simulink model "TP6_Verifcation_intervalle_avec_variables_locales"  (R2022b)
settings: Solver=VariableStepAuto  StartTime=0.0  StopTime=inf  RelTol=1e-3
settings Model: Creator=LENOVO  LastModifiedBy=HP
settings OptimizationCC: ReuseModelBlockBuffer=on
settings RTWCC: GPUComputeCapability=5.0

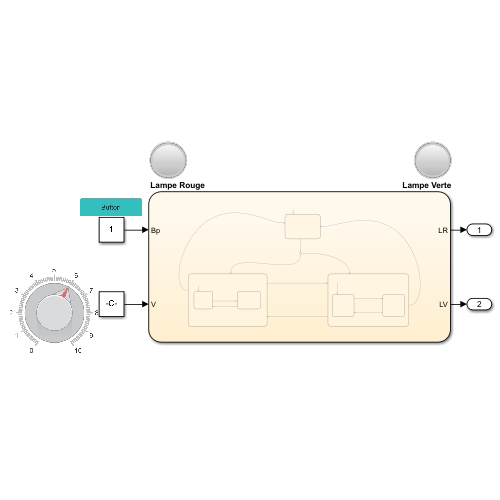
[thumbnail: Simulink's stored preview of the top-level diagram]
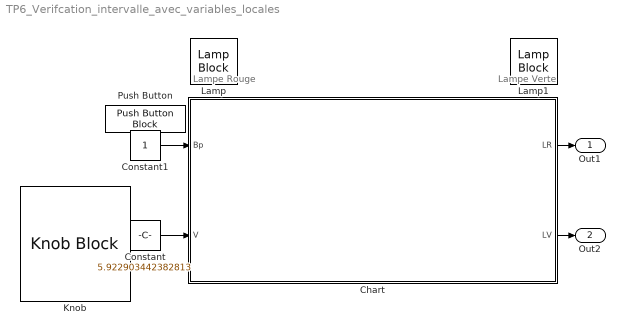
== system TP6_Verifcation_intervalle_avec_variables_locales ==
  note: Lampe Rouge
  note: Lampe Verte
  Chart : Stateflow chart  TreatAsAtomicUnit=on
  Constant : Constant  Value=5.922903442382813
  Constant1 : Constant
  Knob : KnobBlock  LabelPosition=Hide  ScaleMax=10
  Lamp : LampBlock  LabelPosition=Hide
  Lamp1 : LampBlock  LabelPosition=Hide
  Push Button : PushButtonBlock  ButtonType=Latch  OffValue=0.000000
  Out1 : Outport
  Out2 : Outport  Port=2
  wires:
  Constant1/1 -> Chart/1(Bp)
  Constant/1 -> Chart/2(V)
  Chart/1(LR) -> Out1/1
  Chart/2(LV) -> Out2/1

== stateflow chart TP6_Verifcation_intervalle_avec_variables_locales/Chart ==
  state initial
    entry:
    LV=0;
    LR=0;
  state plage_valide
    state on
      entry:
      LV=0;
      LR=1;
    state off
      entry:
      LV=0;
      LR=0;
    (default) -> plage_valide.on
    plage_valide.on -> plage_valide.off : [after (0.5, sec)]
    plage_valide.off -> plage_valide.on : [after (0.5, sec)]
  state plage_invalide
    state on
      entry:
      LV=1;
      LR=0;
    state off
      entry:
      LV=0;
      LR=0;
    (default) -> plage_invalide.on
    plage_invalide.on -> plage_invalide.off : [after (0.5, sec)]
    plage_invalide.off -> plage_invalide.on : [after (0.5, sec)]
  (default) -> initial
  plage_valide -> initial [order 2] : [Bp==0]
  plage_invalide -> initial [order 2] : [Bp==0]
  initial -> (junction 24) : [Bp==1]
  (junction 24) -> plage_invalide [order 2] : [V < A1 || V > A2]
  (junction 24) -> plage_valide [order 1] : [V >= A1 && V <= A2]
  plage_valide -> plage_invalide [order 1] : [Bp==1 && ( V < A1 || V > A2 )]
  plage_invalide -> plage_valide [order 1] : [Bp==1 && ( V >= A1 && V <= A2 )]
  data: A1 local =4; A2 local =7; Bp input; V input; LR output; LV output
